simulink model "Backstepping_SFunction"  (R2021a)
settings: Solver=VariableStepAuto  StartTime=0.0  StopTime=10.0  RelTol=1e-3
settings Model: Creator=45276  LastModifiedBy=45276

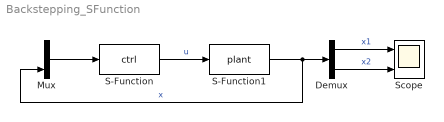
== system Backstepping_SFunction ==
  Demux : Demux  Outputs=2
  Mux : Mux  Inputs=2
  S-Function : S-Function  FunctionName=ctrl  Parameters=pa  SFunctionDeploymentMode=off  EnableBusSupport=off
  S-Function1 : S-Function  FunctionName=plant  Parameters=pa  SFunctionDeploymentMode=off  EnableBusSupport=off
  Scope : Scope  NumInputPorts=2
  wires:
  S-Function/1 -> S-Function1/1  "u"
  S-Function1/1 -> Mux/2, Demux/1  "x"
  Demux/1 -> Scope/1  "x1"
  Demux/2 -> Scope/2  "x2"
  Mux/1 -> S-Function/1
